simulink subsystem "Inputs_MotorDriveUnit_LookupTable_refsub"  (R2026a)
settings: Solver=VariableStepAuto
undefined symbols (not defined in the file or in its folder): MDU_HarnessInputs
libraries: simulink x1
settings Model: Creator=isaacito  LastModifiedBy=ythvg

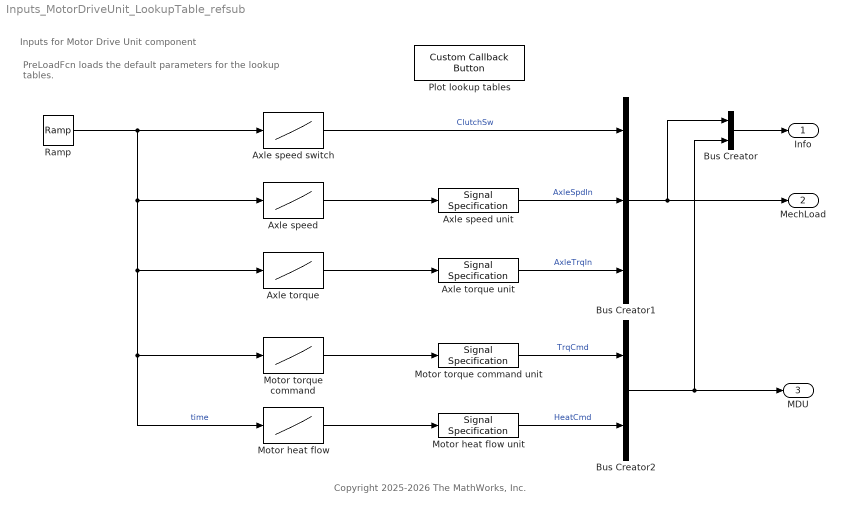
== system Inputs_MotorDriveUnit_LookupTable_refsub ==
  note: Copyright 2025-2026 The MathWorks, Inc.
  note: PreLoadFcn loads the default parameters
      | for the lookup tables.
  note: Inputs for Motor Drive Unit component
  Axle speed : Lookup_n-D  NumberOfTableDimensions=1  BreakpointsForDimension1="MDU_HarnessInputs.AxleSpeed.Time.value(\"s\")"  Table="MDU_HarnessInputs.AxleSpeed.Data.value(\"rpm\")"  InterpMethod=Akima spline  InternalRulePriority=Speed  RndMeth=Simplest
      settings: AttributesFormatString=%<Table>
  Axle speed switch : Lookup_n-D  NumberOfTableDimensions=1  BreakpointsForDimension1="MDU_HarnessInputs.AxleSpeedSwitch.Time.value(\"s\")"  Table=MDU_HarnessInputs.AxleSpeedSwitch.StepValues  InterpMethod=Flat  InternalRulePriority=Speed  RndMeth=Simplest
  Axle speed unit : SignalSpecification  Unit=rpm
  Axle torque : Lookup_n-D  NumberOfTableDimensions=1  BreakpointsForDimension1="MDU_HarnessInputs.AxleTorque.Time.value(\"s\")"  Table="MDU_HarnessInputs.AxleTorque.Data.value(\"N*m\")"  InterpMethod=Akima spline  InternalRulePriority=Speed  RndMeth=Simplest
      settings: AttributesFormatString=%<Table>
  Axle torque unit : SignalSpecification  Unit=N*m
  Bus Creator : BusCreator  Inputs=2
  Bus Creator1 : BusCreator  Inputs=3
  Bus Creator2 : BusCreator  Inputs=2
  Motor heat flow : Lookup_n-D  NumberOfTableDimensions=1  BreakpointsForDimension1="MDU_HarnessInputs.MotorHeatFlow.Time.value(\"s\")"  Table="MDU_HarnessInputs.MotorHeatFlow.Data.value(\"W\")"  InterpMethod=Akima spline  InternalRulePriority=Speed  RndMeth=Simplest
      settings: AttributesFormatString=%<Table>
  Motor heat flow unit : SignalSpecification  Unit=W
  Motor torque command : Lookup_n-D  NumberOfTableDimensions=1  BreakpointsForDimension1="MDU_HarnessInputs.MotorTorqueCommand.Time.value(\"s\")"  Table="MDU_HarnessInputs.MotorTorqueCommand.Data.value(\"N*m\")"  InterpMethod=Akima spline  InternalRulePriority=Speed  RndMeth=Simplest
      settings: AttributesFormatString=%<Table>
  Motor torque command unit : SignalSpecification  Unit=N*m
  Plot lookup tables : CustomCallbackButton  Configuration="{\"components\":[{\"name\":\"BackgroundImageComponent\",\"settings\":{\"image\":{\"size\":[0,0],\"src\":\"default\",\"srcOrientation\":\"Right\"},\"position\":[0,0,1,1]}},{\"name\":\"ButtonStateComponent\",\"settings\":{\"buttonType\":\"momentary\",\"clickFcn\":\"% Specify blocks to sort plot order.\\nblocks = [\\n  \\\"Axle speed switch\\\"\\n  \\\"Axle speed\\\"\\n  \\\"Axle torque\\\"\\n  \\\"Motor torque command\\\"\\n  \\\"Motor heat flow\\\"\\n];\\nbevutil1.SignalUtil.plotLookupTable1DBlocks(gcs, Blocks=blocks, DivisionType=\\\"InterpolationInterval\\\", InterpolationInterval=0.1)\",\"onValue\":1,\"position\":[0,0,1,1],\"pressDelay\":\"500\",\"pressFcn\":\"\",\"repeatInterval\":\"0\",\"states\":[{\"horizontalAlignment\":\"center\",\"image\":{\"position\":[0,0,1,1],\"size\":[1,1],\"src\":\"default\",\"srcOrientation\":\"Right\"},\"label\":{\"color\":[0.01176470588,0.01176470588,0.01176470588,1],\"icon\":{\"size\":[0,0],\"src\":\"default\",\"srcOrientation\":\"Right\"},\"iconOffset\":0,\"iconPlacement\":\"left\",\"opacity\":1,\"show\":true,\"text\":{\"content\":\"Plot LUTs\",\"font\":\"Helvetica\"}},\"labelOffset\":[0,0],\"verticalAlignment\":\"middle\"},{\"horizontalAlignment\":\"center\",\"image\":{\"position\":[0,0,1,1],\"size\":[1,1],\"src\":\"default\",\"srcOrientation\":\"Right\"},\"label\":{\"color\":[0.01176470588,0.01176470588,0.01176470588,1],\"icon\":{\"size\":[0,0],\"src\":\"default\",\"srcOrientation\":\"Right\"},\"iconOffset\":0,\"iconPlacement\":\"left\",\"opacity\":1,\"show\":true,\"text\":{\"content\":\"Plot LUTs\",\"font\":\"Helvetica\"}},\"labelOffset\":[0,0],\"verticalAlignment\":\"middle\"},{\"horizontalAlignment\":\"center\",\"image\":{\"position\":[0,0,1,1],\"size\":[1,1],\"src\":\"default\",\"srcOrientation\":\"Right\"},\"label\":{\"color\":[0.01176470588,0.01176470588,0.01176470588,1],\"icon\":{\"size\":[0,0],\"src\":\"default\",\"srcOrientation\":\"Right\"},\"iconOffset\":0,\"iconPlacement\":\"left\",\"opacity\":1,\"show\":true,\"text\":{\"content\":\"Plot LUTs\",\"font\":\"Helvetica\"}},\"labelOffset\":[0,0],\"verticalAlignment\":\"middle\"},{\"horizontalAlignment\":\"center\",\"image\":{\"position\":[0,0,1,1],\"size\":[1,1],\"src\":\"default\",\"srcOrientation\":\"Right\"},\"label\":{\"color\":[0.01176470588,0.01176470588,0.01176470588,1],\"icon\":{\"size\":[0,0],\"src\":\"default\",\"srcOrientation\":\"Right\"},\"iconOffset\":0,\"iconPlacement\":\"left\",\"opacity\":1,\"show\":true,\"text\":{\"content\":\"Plot LUTs\",\"font\":\"Helvetica\"}},\"labelOffset\":[0,0],\"verticalAlignment\":\"middle\"}]}},{\"name\":\"ForegroundImageComponent\",\"settings\":{\"image\":{\"size\":[0,0],\"src\":\"default\",\"srcOrientation\":\"Right\"},\"isForeground\":1,\"position\":[0,0,1,1]}}],\"derived\":{\"blockParameters\":{\"AutoActivate\":true,\"ButtonText\":\"Plot LUTs\",\"ButtonType\":\"Momentary\",\"ClickFcn\":\"% Specify blocks to sort plot order.\\nblocks = [\\n  \\\"Axle speed switch\\\"\\n  \\\"Axle speed\\\"\\n  \\\"Axle torque\\\"\\n  \\\"Motor torque command\\\"\\n  \\\"Motor heat flow\\\"\\n];\\nbevutil1.SignalUtil.plotLookupTable1DBlocks(gcs, Blocks=blocks, DivisionType=\\\"InterpolationInterval\\\", InterpolationInterval=0.1)\",\"OnValue\":1,\"PressDelay\":\"500\",\"PressFcn\":\"\",\"RepeatInterval\":\"0\",\"fixedAspectRatio\":\"off\"}},\"settings\":{\"BindingType\":\"standalone\",\"autoActivate\":true,\"backgroundColor\":[244,244,244,1],\"backgroundOffset\":0.2,\"backgroundOpacity\":1,\"fixedAspectRatio\":\"off\",\"foregroundColor\":[0.01176470588,0.01176470588,0.01176470588,1],\"migratedFromLegacy\":true,\"useBackgroundColor\":true,\"variant\":\"callback\",\"version\":\"R2025a\"},\"type\":\"Button\"}"  CustomBackgroundColor="{\"color\":[0.9568627451,0.9568627451,0.9568627451],\"show\":true}"
  Ramp : simulink/Sources/Ramp  slope=1  start=0  InitialOutput=0
      settings: AttributesFormatString=|
      | Slope: %<slope>
      | Start time: %<start>
      | Initial output: %<InitialOutput>
  Info : Outport
  MechLoad : Outport  Port=2
  MDU : Outport  Port=3
  wires:
  Bus Creator/1 -> Info/1
  Motor torque command unit/1 -> Bus Creator2/1  "TrqCmd"
  Axle torque unit/1 -> Bus Creator1/3  "AxleTrqIn"
  Axle speed unit/1 -> Bus Creator1/2  "AxleSpdIn"
  Motor heat flow unit/1 -> Bus Creator2/2  "HeatCmd"
  Bus Creator2/1 -> Bus Creator/2, MDU/1
  Bus Creator1/1 -> Bus Creator/1, MechLoad/1
  Ramp/1 -> Axle speed switch/1, Axle speed/1, Axle torque/1, Motor heat flow/1, Motor torque command/1  "time"
  Axle speed switch/1 -> Bus Creator1/1  "ClutchSw"
  Axle speed/1 -> Axle speed unit/1
  Axle torque/1 -> Axle torque unit/1
  Motor torque command/1 -> Motor torque command unit/1
  Motor heat flow/1 -> Motor heat flow unit/1
